simulink model "ECP_InvertedPendulum"  (R2025a)
settings: Solver=VariableStepAuto  StartTime=0.0  StopTime=100  RelTol=1e-3
values from neighbouring files (symbols this model uses):
  g = 9.807    [SlidingRodPendulum_Modeling.m]
  J_oe = J_star_o + m_1*l_o^2 + m_w2*l_w2^2    (= 0.05954626)    [SlidingRodPendulum_Modeling.m]
  J_star = J_oe-m_1*l_o^2    (= 0.03635056)    [SlidingRodPendulum_Modeling.m]
  k_a = 2546    [SlidingRodPendulum_Modeling.m]
  k_f = 0.0013    [SlidingRodPendulum_Modeling.m]
  k_pfc = S0+R0/G2_dc    [SlidingRodPendulum_Modeling.m]
  k_s = 32    [SlidingRodPendulum_Modeling.m]
  k_x = 50200    [SlidingRodPendulum_Modeling.m]
  kd = 2*zeta*wn*m_star/k_hw    (= 0.00784530292237)    [SlidingRodPendulum_Modeling.m]
  kp = m_star*wn^2/k_hw    (= 0.247127042055)    [SlidingRodPendulum_Modeling.m]
  l_c = (m_w2*l_w2+m_2o*l_co)/(m_2)    (= -0.0294602240896)    [SlidingRodPendulum_Modeling.m]
  l_o = 0.330    (= 0.33)    [SlidingRodPendulum_Modeling.m]
  m_1 = m_1o+m_w1    (= 0.213)    [SlidingRodPendulum_Modeling.m]
  m_2 = m_2o+m_w2    (= 1.785)    [SlidingRodPendulum_Modeling.m]
  r_0_val = double(sol.r_0)    [SlidingRodPendulum_Modeling.m]
  r_1_val = double(sol.r_1)    [SlidingRodPendulum_Modeling.m]
  s_0_val = double(sol.s_0)    [SlidingRodPendulum_Modeling.m]
  s_1_val = double(sol.s_1)    [SlidingRodPendulum_Modeling.m]
libraries: slpidlib x1, simulink_extras x1
settings Model: Creator=young  LastModifiedBy=young
settings DataIOCC: ReturnWorkspaceOutputs=off

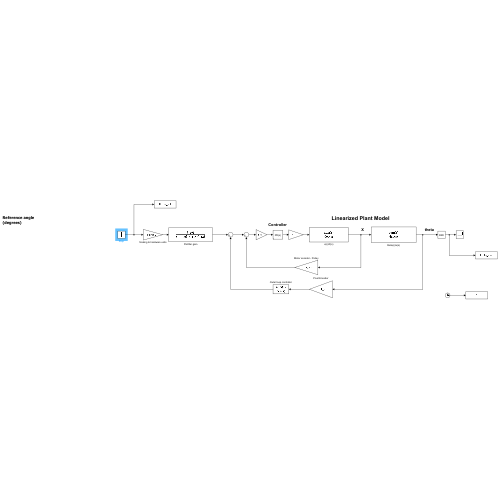
[thumbnail: Simulink's stored preview of the top-level diagram]
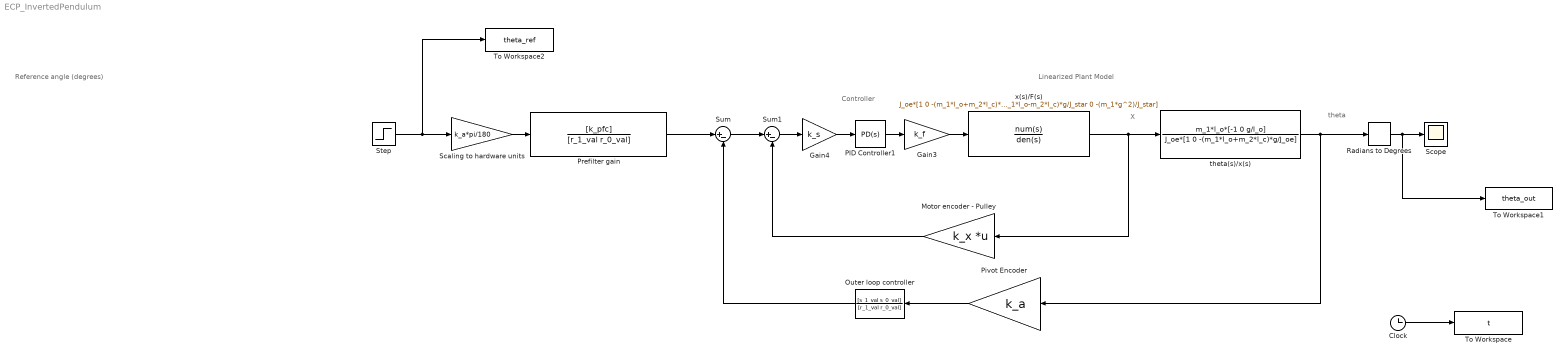
== system ECP_InvertedPendulum ==
  note: Reference angle (degrees)
  note: Controller
  note: theta
  note: X
  note: Linearized Plant Model
  Clock : Clock
  Gain3 : Gain  Gain=k_f
  Gain4 : Gain  Gain=k_s
  Motor encoder - Pulley : Gain  Gain=k_x  Multiplication=Matrix(K*u)
  Outer loop controller : TransferFcn  Numerator=[s_1_val s_0_val]  Denominator=[r_1_val r_0_val]
  PID Controller1 : slpidlib/PID Controller  Controller=PD  Form=Parallel  TimeDomain=Continuous-time  UseExternalTs=off  SampleTime=-1  IntegratorMethod=Forward Euler  FilterMethod=Forward Euler  ControllerParametersSource=internal  P=kp  I=0  UseKiTs=off  D=kd  UseExternalDerivativeSource=off  N=100  UseFilter=on  TunerSelectOption=Transfer Function Based (PID Tuner App)  InitialConditionSource=internal  InitialConditionForIntegrator=0  InitialConditionForFilter=0  DifferentiatorICPrevScaledInput=0  ExternalReset=none  TrackingMode=off  Kt=1  LimitOutput=off  SatLimitsSource=internal  UpperSaturationLimit=inf  LowerSaturationLimit=-inf  LinearizeAsGain=on  AntiWindupMode=none  Kb=1  LimitIntegrator=off  UpperIntegratorSaturationLimit=inf  LowerIntegratorSaturationLimit=-inf  POutMin=[]  POutMax=[]  IOutMin=[]  IOutMax=[]  DOutMin=[]  DOutMax=[]  NOutMin=[]  NOutMax=[]  SumOutMin=[]  SumOutMax=[]  SaturationOutMin=[]  SaturationOutMax=[]  PParamMin=[]  PParamMax=[]  IParamMin=[]  IParamMax=[]  DParamMin=[]  DParamMax=[]  NParamMin=[]  NParamMax=[]  KbParamMin=[]  KbParamMax=[]  KtParamMin=[]  KtParamMax=[]  KbOutMin=[]  KbOutMax=[]  KtOutMin=[]  KtOutMax=[]  IntegratorOutMin=[]  IntegratorOutMax=[]  FilterOutMin=[]  FilterOutMax=[]  SumI1OutMin=[]  SumI1OutMax=[]  SumI2OutMin=[]  SumI2OutMax=[]  SumI3OutMin=[]  SumI3OutMax=[]  SumI4OutMin=[]  SumI4OutMax=[]  SumDOutMin=[]  SumDOutMax=[]  DifferentiatorOutMin=[]  DifferentiatorOutMax=[]  FilterDiffOutCoefMin=[]  FilterDiffOutCoefMax=[]  ReciprocalOutMin=[]  ReciprocalOutMax=[]  SumDenOutMin=[]  SumDenOutMax=[]  SumNumOutMin=[]  SumNumOutMax=[]  DivideOutMin=[]  DivideOutMax=[]  UdiffTsProdOutMin=[]  UdiffTsProdOutMax=[]  NTsProdOutMin=[]  NTsProdOutMax=[]  UintegralTsProdOutMin=[]  UintegralTsProdOutMax=[]  UngainTsProdOutMin=[]  UngainTsProdOutMax=[]  ClampingZeroOutDataTypeStr=Inherit: Inherit via back propagation  ClampingZeroOutMin=[]  ClampingZeroOutMax=[]  FilterDenConstantOutDataTypeStr=Inherit: Inherit via back propagation  FilterDenConstantOutMin=[]  FilterDenConstantOutMax=[]  PCopyOutDataTypeStr=Inherit: Inherit via back propagation  PCopyOutMin=[]  PCopyOutMax=[]  NCopyOutDataTypeStr=Inherit: Inherit via back propagation  NCopyOutMin=[]  NCopyOutMax=[]  IntegratorContinuousStateAttributes=''  IntegratorStateMustResolveToSignalObject=off  IntegratorRTWStateStorageClass=Auto  FilterContinuousStateAttributes=''  FilterStateMustResolveToSignalObject=off  FilterRTWStateStorageClass=Auto  ParallelPVariant=InternalParameters  IdealPVariant=Disabled  IVariant=Disabled  DVariant=InternalParameters  IntegratorVariant=Disabled  SatVariant=Disabled  AWVariant=Disabled  PCopyVariant=Disabled  TRVariant=Disabled  FdbkBlocksVariant=Forward  IdealPFdbkVariant=Disabled  SatFdbkVariant=Disabled  DerivativeFilterVariant=ContFilter  NVariant=InternalParameters  NCopyVariant=Disabled  FilterICVariant=InternalICsFilter  IntegratorICVariant=Disabled  ExternalResetVariant=Disabled  TRSumVariant=Passthrough  SumFdbkVariant=Disabled  SumVariant=Sum_PD  TsampFilterVariant=InternalTs  TsampNgainVariant=Passthrough  TsampIntegralVariant=Disabled_SignalSpec  ExternalSaturationOutDataTypeStr=Inherit: Same as second input  DerivativeSourceVariant=ErrorSignal  PreIntVariant=InternalPreInt
  Pivot Encoder : Gain  Gain=k_a
  Prefilter gain : TransferFcn  Numerator=[k_pfc]  Denominator=[r_1_val r_0_val]
  Radians to Degrees : simulink_extras/Transformations/Radians to Degrees
  Scaling to hardware units : Gain  Gain=k_a*pi/180
  Scope : Scope
      settings: ActiveDisplayYMinimum=-10.568448256192054  ActiveDisplayYMaximum=25.551840627087003
  Step : Step  Time=0  After=20  SampleTime=0
  Sum : Sum  Inputs=|+-
  Sum1 : Sum  Inputs=|+-
  To Workspace : ToWorkspace  VariableName=t  SampleTime=-1
  To Workspace1 : ToWorkspace  VariableName=theta_out  SampleTime=-1
  To Workspace2 : ToWorkspace  VariableName=theta_ref  SampleTime=-1
  theta(s)/x(s) : TransferFcn  Numerator=m_1*l_o*[-1 0 g/l_o]  Denominator=J_oe*[1 0 -(m_1*l_o+m_2*l_c)*g/J_oe]
  x(s)/F(s) : TransferFcn  Numerator=J_oe*[1 0 -(m_1*l_o+m_2*l_c)*g/J_oe]  Denominator=m_1*J_star*[1 0 (m_1*l_o-m_2*l_c)*g/J_star 0 -(m_1*g^2)/J_star]
  wires:
  Gain3/1 -> x(s)/F(s)/1
  Sum1/1 -> Gain4/1
  PID Controller1/1 -> Gain3/1
  Gain4/1 -> PID Controller1/1
  x(s)/F(s)/1 -> theta(s)/x(s)/1, Motor encoder - Pulley/1
  theta(s)/x(s)/1 -> Radians to Degrees/1, Pivot Encoder/1
  Motor encoder - Pulley/1 -> Sum1/2
  Pivot Encoder/1 -> Outer loop controller/1
  Prefilter gain/1 -> Sum/1
  Outer loop controller/1 -> Sum/2
  Step/1 -> To Workspace2/1, Scaling to hardware units/1
  Sum/1 -> Sum1/1
  Scaling to hardware units/1 -> Prefilter gain/1
  Radians to Degrees/1 -> To Workspace1/1, Scope/1
  Clock/1 -> To Workspace/1
